simulink model "Dock_Charger"  (R2026b)
settings: Solver=VariableStepAuto
undefined symbols (not defined in the file or in its folder): P, Ts
libraries: nesl_utility x7, ee_lib x6, fl_lib x5, simulink x2, eeGeneralControl x1, batt_lib x1
settings Model: Creator=aomar  LastModifiedBy=aomar

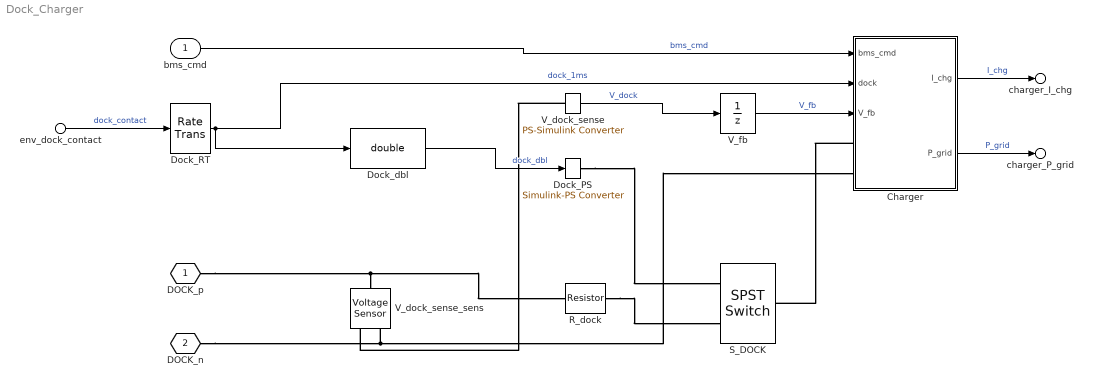
== system Dock_Charger ==
  bms_cmd : Inport  OutDataTypeStr=Bus: Bus_BMS_Cmd  SampleTime=Ts.bms_fast
  env_dock_contact : Inport  Port=2  PortName=env  Element=dock_contact
  Charger : Subsystem  Variant=on
  Dock_PS : nesl_utility/Simulink-PS Converter  PhysicalDomain=network_engine_domain  SubClassName=ps_input  LeftPortType=input  RightPortType=output  PseudoPeriodic=off  Frequencies=[]  NoiseDistribution=none  NoiseParameters=[]  Unit=V  AffineConversion=off  FilteringAndDerivatives=zero  SimscapeFilterOrder=1  InputFilterTimeConstant=0.001  UdotUserProvided=0
  Dock_RT : RateTransition  OutPortSampleTime=Ts.base
  Dock_dbl : DataTypeConversion  OutDataTypeStr=double  SaturateOnIntegerOverflow=off  RndMeth=Floor
  R_dock : ee_lib/Passive/Resistor  R=P.power.charger.R_dock Ohm  enable_R_tol=ee.enum.toleranceApplication.none  R_tol=5  tol_distribution=ee.enum.toleranceDistribution.uniform  nSigma=4  enable_operating_limits=ee.enum.enable.no  operating_limit_action=ee.enum.passive.reportOpLim.warn  power_rating=1 W  max_working_voltage=100 V  noise_mode=ee.enum.sources.noise.Disabled  Tdevice=25 degC  sample_time=1e-3 s  repeatability=ee.enum.ic.repeatability.notRepeatable  user_seed=0  auto_seed=1684602222  power_derating_T1=70 degC  power_derating_T2=155 degC  operating_temperature_range_vec=[-50, 150] degC  alpha=3.93e-3 1/K  Tmeas=25 degC  thermal_mass=100 J/K  temperature_specify=off  temperature_priority=High  temperature=298.15 K  temperature_nominal_specify=off  temperature_nominal_value=1  temperature_nominal_unit=K
  S_DOCK : ee_lib/Switches & Breakers/SPST Switch  R_closed=1e-6 Ohm  G_open=1e-8 S  Threshold=0.5 V  Width=0 V  model_dynamics=0  t_on=1e-3 s  t_off=1e-3 s  initial_vT=0 V
  V_dock_sense : nesl_utility/PS-Simulink Converter  PhysicalDomain=network_engine_domain  SubClassName=ps_output  LeftPortType=input  RightPortType=output  PseudoPeriodic=off  Frequencies=[]  VectorFormat=inherit  Unit=V  AffineConversion=off
  V_dock_sense_sens : fl_lib/Electrical/Electrical Sensors/Voltage Sensor
  V_fb : UnitDelay  SampleTime=Ts.base
  DOCK_p : PMIOPort  Side=Left  ConnectionType=Connection: foundation.electrical.electrical
  DOCK_n : PMIOPort  Port=2  Side=Left  ConnectionType=Connection: foundation.electrical.electrical
  charger_P_grid : Outport  PortName=charger  Element=P_grid
  charger_I_chg : Outport  PortName=charger  Element=I_chg
  wires:
  env_dock_contact/1 -> Dock_RT/1  "dock_contact"
  bms_cmd/1 -> Charger/1(bms_cmd)  "bms_cmd"
  Dock_RT/1 -> Charger/2(dock), Dock_dbl/1  "dock_1ms"
  Dock_dbl/1 -> Dock_PS/1  "dock_dbl"
  V_dock_sense/1 -> V_fb/1  "V_dock"
  V_fb/1 -> Charger/3(V_fb)  "V_fb"
  Charger/1(I_chg) -> charger_I_chg/1  "I_chg"
  Charger/2(P_grid) -> charger_P_grid/1  "P_grid"
  connections:
  Charger/LConn1 -- S_DOCK/RConn1
  V_dock_sense_sens/RConn2 -- DOCK_n/RConn1 -- Charger/LConn2
  V_dock_sense_sens/LConn1 -- DOCK_p/RConn1 -- R_dock/LConn1
  Dock_PS/RConn1 -- S_DOCK/LConn1
  R_dock/RConn1 -- S_DOCK/LConn2
  V_dock_sense/LConn1 -- V_dock_sense_sens/RConn1

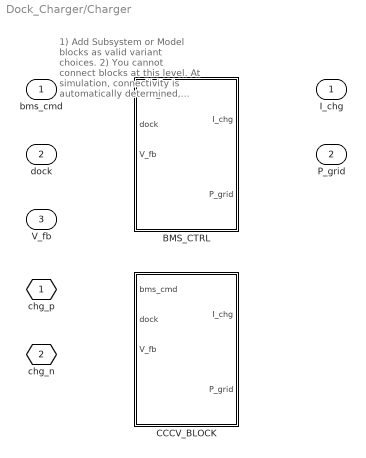
== system Dock_Charger/Charger ==
  note: 1) Add Subsystem or Model blocks as valid variant choices.
      | 2) You cannot connect blocks at this level. At simulation, connectivity is automatically
      | determined, based on the active variant and port name matching.
  bms_cmd : Inport
  dock : Inport  Port=2
  V_fb : Inport  Port=3
  BMS_CTRL : Subsystem  VariantControl=VC_CHG == 1
  CCCV_BLOCK : Subsystem  VariantControl=VC_CHG == 2
  chg_p : PMIOPort  Side=Left  ConnectionType=Connection: foundation.electrical.electrical
  chg_n : PMIOPort  Port=2  Side=Left  ConnectionType=Connection: foundation.electrical.electrical
  I_chg : Outport
  P_grid : Outport  Port=2

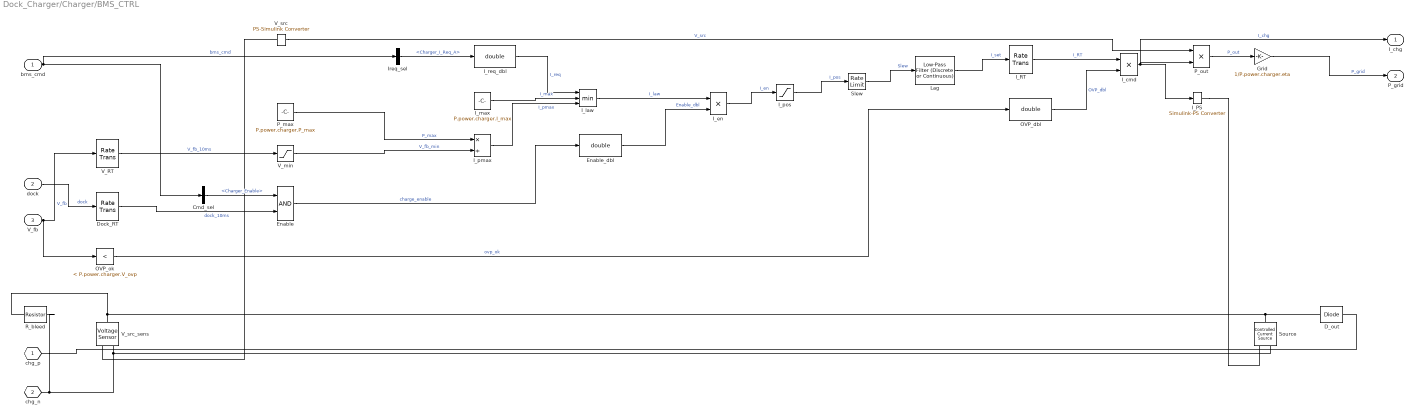
== system Dock_Charger/Charger/BMS_CTRL ==
  bms_cmd : Inport
  dock : Inport  Port=2
  V_fb : Inport  Port=3
  Cmd_sel : BusSelector  OutputSignals=Charger_Enable
  D_out : ee_lib/Semiconductors & Converters/Diode  Vf=P.power.charger.diode_Vf V  Ron=P.power.charger.diode_Ron Ohm  Goff=P.power.charger.diode_Goff S  N_series=1  N_parallel=1  ZenerEnable=false  BV=30 V  Rz=0.3 Ohm  enable_fault_composite=simscape.enum.onoff.off  i_specify=off  i_priority=None  i=0 A  i_nominal_specify=off  i_nominal_value=1  i_nominal_unit=A  v_specify=off  v_priority=None  v=0 V  v_nominal_specify=off  v_nominal_value=1  v_nominal_unit=V  ModelType=ee.enum.diode.idealModelType.pwl  TableType=ee.enum.diode.tableType.IfMat  IfMat=[.07, .12, .19, 1.75, 4.24, 7.32, 11.2; .16, .3, .72, 2.14, 5.02, 8.35, 13.12] A  VfMat=[.9, 1.15, 1.25, 1.5, 1.75, 2.17, 2.6, 2.85; .58, .68, .75, 1.1, 1.38, 1.77, 2.27, 2.7] V  TjVec=[25, 125] degC  VfVec=[.5, .7, .9, 1.3, 1.7, 2.1, 2.5] V  IfVec=[.1, .2, .5, 1, 2, 4, 7, 10] A  IrMat=[1e-06, 2e-06, 5e-06, 1e-05, 2.5e-05, 5e-05, .0001; 2e-06, 5e-06, 1e-05, 4e-05, 8e-05, .0002, .0005] A  VrMat=[10, 100, 200, 250, 300, 325, 350; 10, 70, 160, 220, 270, 300, 320] V  VrVec=[10, 20, 40, 50, 70, 80, 100] V  IrVec=[1e-06, 2e-06, 5e-06, 1e-05, 2e-05, 5e-05, .0001] A  rec_loss_model=ee.enum.diode.reverseRecoveryModelTabulateUpTo3D.fixed  ErecVal=0 J  scaleWithIandV=true  ErecMat=zeros(2, 3) J  ErecMat3D=zeros(2, 3, 2) J  TjrecVec=[25, 125] degC  IfrecVec=[.1, 1, 10] A  IrecVal=10 A  VrecVal=10 V  VrecVec=[0, 100] V  tFilter=1 / 1000 / 100 s  thermal_network_parameterization=ee.enum.thermalNetworkTopology.junctionCase  Rth=[0, 10] K/W  Rth_Cauer=[1, 3, 10] K/W  Rth_Foster=[.08, .14, .22, .16] K/W  thermal_mass_parameterization=ee.enum.thermalNetwork.timeconstant  thermal_mass=[0, 1] J/K  thermal_mass_Cauer=[.1, .3, 1] J/K  thermal_mass_Foster=[.001, .005, .05, .5] J/K  thermal_time_constant=[0, 10] s  thermal_time_constant_Cauer=[1, 3, 10] s  thermal_time_constant_Foster=[7e-05, .0007, .01, .08] s  thermal_mass_initial_temperatures=[25, 25] degC  thermal_mass_initial_temperatures_Cauer=[25, 25, 25] degC  thermal_mass_initial_temperatures_Foster=[25, 25, 25, 25] degC  junction_thermal_mass=0.01 J/K  junction_temperature_specify=off  junction_temperature_priority=None  junction_temperature=25 degC  junction_temperature_nominal_specify=off  junction_temperature_nominal_value=1  junction_temperature_nominal_unit=degC  ThermalPort=false  ModelTypePhysical=ee.enum.diode.physicalModelType.exponential  prmExp=ee.enum.diode.expParam.useTwo  I12=[.0137, .545] A  V12=[.6, .7] V  IS=1e-12 A  ec=1  I1=0.0137 A  V1=0.6 V  RS=0 Ohm  C_param=ee.enum.diode.capParam.fixed  CJ=0 pF  CJ0=5 pF  Vvec=[.1, 10, 100] V  Cvec=[3.5, 1, .4] pF  VJ=1 V  Mgrad=0.5  FC=0.5  Q_param=ee.enum.diode.recoveryParam.off  iRM=-7.15 A  iF=4 A  didt=-750 A/us  trr_factor=3  trr=115 ns  Qrr=150 nA*s  Vr=-600 V  Ls=150 nH  Erec=0.03 J  TT=50 ns  tau=100 ns  T_param=ee.enum.diode.temperatureParam.off  Tmeas=25 degC  I1_T2=0.245 A  V1_T2=0.5 V  IS_T2=1.25e-7 A  Tmeas2=125 degC  EG_param=ee.enum.diode.egapParam.material_si  EG=1.11 eV  XTI_param=ee.enum.diode.xtiParam.pn  XTI=3  dBVdT=0 V/K  Tdevice=25 degC  i_capacitor_specify=off  i_capacitor_priority=None  i_capacitor=0 A  i_capacitor_nominal_specify=off  i_capacitor_nominal_value=1  i_capacitor_nominal_unit=A  Qj_specify=off  Qj_priority=None  Qj=0 C  Qj_nominal_specify=off  Qj_nominal_value=1  Qj_nominal_unit=uC
  Dock_RT : RateTransition  OutPortSampleTime=Ts.bms_fast
  Enable : Logic  AllPortsSameDT=off  OutDataTypeStr=boolean
  Enable_dbl : DataTypeConversion  OutDataTypeStr=double  SaturateOnIntegerOverflow=off  RndMeth=Floor
  Grid : Gain  Gain=1/P.power.charger.eta
  I_PS : nesl_utility/Simulink-PS Converter  PhysicalDomain=network_engine_domain  SubClassName=ps_input  LeftPortType=input  RightPortType=output  PseudoPeriodic=off  Frequencies=[]  NoiseDistribution=none  NoiseParameters=[]  Unit=A  AffineConversion=off  FilteringAndDerivatives=zero  SimscapeFilterOrder=1  InputFilterTimeConstant=0.001  UdotUserProvided=0
  I_RT : RateTransition  OutPortSampleTime=Ts.base
  I_cmd : Product
  I_en : Product
  I_law : MinMax  Inputs=3
  I_max : Constant  Value=P.power.charger.I_max  SampleTime=Ts.bms_fast
  I_pmax : Product  Inputs=*/
  I_pos : Saturate  UpperLimit=inf  LowerLimit=0
  I_req_dbl : DataTypeConversion  OutDataTypeStr=double  SaturateOnIntegerOverflow=off  RndMeth=Floor
  Ireq_sel : BusSelector  OutputSignals=Charger_I_Req_A
  Lag : eeGeneralControl/Low-Pass Filter (Discrete or Continuous)  K=1  T=P.power.charger.tau  B=inf  A=-inf  init_option=Specify as parameter  x0=0  Ts=Ts.bms_fast
  OVP_dbl : DataTypeConversion  OutDataTypeStr=double  SaturateOnIntegerOverflow=off  RndMeth=Floor
  OVP_ok : simulink/Logic and Bit Operations/Compare To Constant  relop=<  const=P.power.charger.V_ovp  OutDataTypeStr=boolean
  P_max : Constant  Value=P.power.charger.P_max  SampleTime=Ts.bms_fast
  P_out : Product
  R_bleed : ee_lib/Passive/Resistor  R=P.power.charger.R_bleed Ohm  enable_R_tol=ee.enum.toleranceApplication.none  R_tol=5  tol_distribution=ee.enum.toleranceDistribution.uniform  nSigma=4  enable_operating_limits=ee.enum.enable.no  operating_limit_action=ee.enum.passive.reportOpLim.warn  power_rating=1 W  max_working_voltage=100 V  noise_mode=ee.enum.sources.noise.Disabled  Tdevice=25 degC  sample_time=1e-3 s  repeatability=ee.enum.ic.repeatability.notRepeatable  user_seed=0  auto_seed=2815256101  power_derating_T1=70 degC  power_derating_T2=155 degC  operating_temperature_range_vec=[-50, 150] degC  alpha=3.93e-3 1/K  Tmeas=25 degC  thermal_mass=100 J/K  temperature_specify=off  temperature_priority=High  temperature=298.15 K  temperature_nominal_specify=off  temperature_nominal_value=1  temperature_nominal_unit=K
  Slew : RateLimiter  RisingSlewLimit=P.power.charger.slew  FallingSlewLimit=-P.power.charger.slew  SampleTimeMode=inherited
  Source : fl_lib/Electrical/Electrical Sources/Controlled Current Source
  V_RT : RateTransition  OutPortSampleTime=Ts.bms_fast
  V_min : Saturate  UpperLimit=inf  LowerLimit=1
  V_src : nesl_utility/PS-Simulink Converter  PhysicalDomain=network_engine_domain  SubClassName=ps_output  LeftPortType=input  RightPortType=output  PseudoPeriodic=off  Frequencies=[]  VectorFormat=inherit  Unit=V  AffineConversion=off
  V_src_sens : fl_lib/Electrical/Electrical Sensors/Voltage Sensor
  chg_p : PMIOPort  Side=Left  ConnectionType=Connection: foundation.electrical.electrical
  chg_n : PMIOPort  Port=2  Side=Left  ConnectionType=Connection: foundation.electrical.electrical
  I_chg : Outport
  P_grid : Outport  Port=2
  wires:
  bms_cmd/1 -> Cmd_sel/1, Ireq_sel/1  "bms_cmd"
  dock/1 -> Dock_RT/1  "dock"
  V_fb/1 -> V_RT/1, OVP_ok/1  "V_fb"
  OVP_ok/1 -> OVP_dbl/1  "ovp_ok"
  V_RT/1 -> V_min/1  "V_fb_10ms"
  Dock_RT/1 -> Enable/2  "dock_10ms"
  Cmd_sel/1 -> Enable/1  "<Charger_Enable>"
  V_src/1 -> P_out/1  "V_src"
  P_max/1 -> I_pmax/1  "P_max"
  V_min/1 -> I_pmax/2  "V_fb_min"
  Enable/1 -> Enable_dbl/1  "charge_enable"
  Ireq_sel/1 -> I_req_dbl/1  "<Charger_I_Req_A>"
  I_max/1 -> I_law/2  "I_max"
  I_pmax/1 -> I_law/3  "I_pmax"
  I_req_dbl/1 -> I_law/1  "I_req"
  I_law/1 -> I_en/1  "I_law"
  Enable_dbl/1 -> I_en/2  "Enable_dbl"
  I_en/1 -> I_pos/1  "I_en"
  I_pos/1 -> Slew/1  "I_pos"
  Slew/1 -> Lag/1  "Slew"
  Lag/1 -> I_RT/1  "I_set"
  I_RT/1 -> I_cmd/1  "I_RT"
  OVP_dbl/1 -> I_cmd/2  "OVP_dbl"
  I_cmd/1 -> I_PS/1, I_chg/1, P_out/2  "I_chg"
  P_out/1 -> Grid/1  "P_out"
  Grid/1 -> P_grid/1  "P_grid"
  connections:
  V_src_sens/LConn1 -- R_bleed/LConn1 -- Source/LConn1 -- D_out/LConn1
  I_PS/RConn1 -- Source/RConn1
  V_src/LConn1 -- V_src_sens/RConn1
  chg_p/RConn1 -- D_out/RConn1
  chg_n/RConn1 -- R_bleed/RConn1 -- V_src_sens/RConn2 -- Source/RConn2

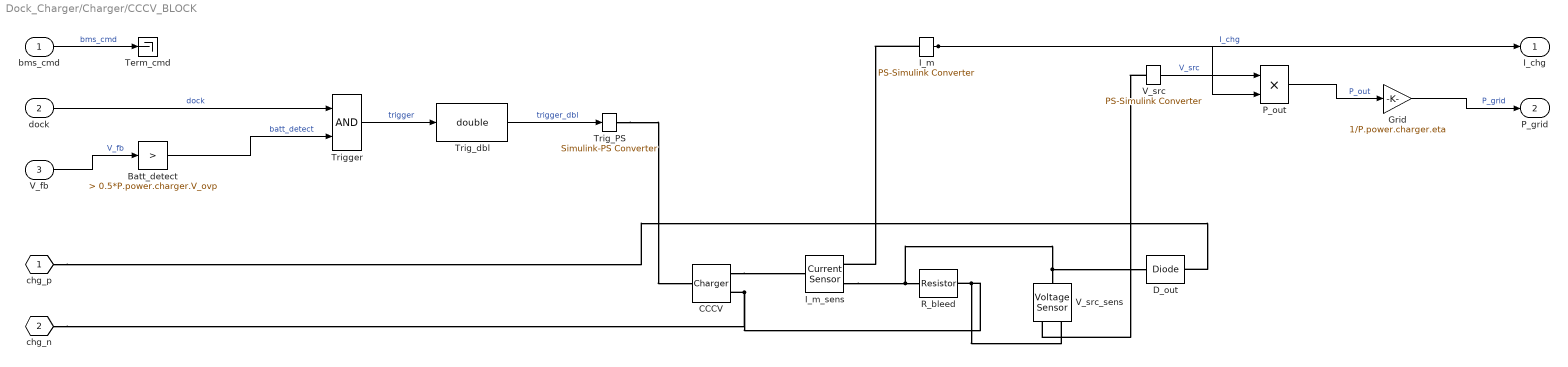
== system Dock_Charger/Charger/CCCV_BLOCK ==
  bms_cmd : Inport
  dock : Inport  Port=2
  V_fb : Inport  Port=3
  Batt_detect : simulink/Logic and Bit Operations/Compare To Constant  relop=>  const=0.5*P.power.charger.V_ovp  OutDataTypeStr=boolean
  CCCV : batt_lib/Cyclers/Charger  charging_current=P.power.charger.cccv_I A  voltage_threshold=P.power.charger.cccv_Vth V  charging_voltage=P.power.charger.cccv_V V  current_threshold=P.power.charger.cccv_Ith A
  D_out : ee_lib/Semiconductors & Converters/Diode  Vf=P.power.charger.diode_Vf V  Ron=P.power.charger.diode_Ron Ohm  Goff=P.power.charger.diode_Goff S  N_series=1  N_parallel=1  ZenerEnable=false  BV=30 V  Rz=0.3 Ohm  enable_fault_composite=simscape.enum.onoff.off  i_specify=off  i_priority=None  i=0 A  i_nominal_specify=off  i_nominal_value=1  i_nominal_unit=A  v_specify=off  v_priority=None  v=0 V  v_nominal_specify=off  v_nominal_value=1  v_nominal_unit=V  ModelType=ee.enum.diode.idealModelType.pwl  TableType=ee.enum.diode.tableType.IfMat  IfMat=[.07, .12, .19, 1.75, 4.24, 7.32, 11.2; .16, .3, .72, 2.14, 5.02, 8.35, 13.12] A  VfMat=[.9, 1.15, 1.25, 1.5, 1.75, 2.17, 2.6, 2.85; .58, .68, .75, 1.1, 1.38, 1.77, 2.27, 2.7] V  TjVec=[25, 125] degC  VfVec=[.5, .7, .9, 1.3, 1.7, 2.1, 2.5] V  IfVec=[.1, .2, .5, 1, 2, 4, 7, 10] A  IrMat=[1e-06, 2e-06, 5e-06, 1e-05, 2.5e-05, 5e-05, .0001; 2e-06, 5e-06, 1e-05, 4e-05, 8e-05, .0002, .0005] A  VrMat=[10, 100, 200, 250, 300, 325, 350; 10, 70, 160, 220, 270, 300, 320] V  VrVec=[10, 20, 40, 50, 70, 80, 100] V  IrVec=[1e-06, 2e-06, 5e-06, 1e-05, 2e-05, 5e-05, .0001] A  rec_loss_model=ee.enum.diode.reverseRecoveryModelTabulateUpTo3D.fixed  ErecVal=0 J  scaleWithIandV=true  ErecMat=zeros(2, 3) J  ErecMat3D=zeros(2, 3, 2) J  TjrecVec=[25, 125] degC  IfrecVec=[.1, 1, 10] A  IrecVal=10 A  VrecVal=10 V  VrecVec=[0, 100] V  tFilter=1 / 1000 / 100 s  thermal_network_parameterization=ee.enum.thermalNetworkTopology.junctionCase  Rth=[0, 10] K/W  Rth_Cauer=[1, 3, 10] K/W  Rth_Foster=[.08, .14, .22, .16] K/W  thermal_mass_parameterization=ee.enum.thermalNetwork.timeconstant  thermal_mass=[0, 1] J/K  thermal_mass_Cauer=[.1, .3, 1] J/K  thermal_mass_Foster=[.001, .005, .05, .5] J/K  thermal_time_constant=[0, 10] s  thermal_time_constant_Cauer=[1, 3, 10] s  thermal_time_constant_Foster=[7e-05, .0007, .01, .08] s  thermal_mass_initial_temperatures=[25, 25] degC  thermal_mass_initial_temperatures_Cauer=[25, 25, 25] degC  thermal_mass_initial_temperatures_Foster=[25, 25, 25, 25] degC  junction_thermal_mass=0.01 J/K  junction_temperature_specify=off  junction_temperature_priority=None  junction_temperature=25 degC  junction_temperature_nominal_specify=off  junction_temperature_nominal_value=1  junction_temperature_nominal_unit=degC  ThermalPort=false  ModelTypePhysical=ee.enum.diode.physicalModelType.exponential  prmExp=ee.enum.diode.expParam.useTwo  I12=[.0137, .545] A  V12=[.6, .7] V  IS=1e-12 A  ec=1  I1=0.0137 A  V1=0.6 V  RS=0 Ohm  C_param=ee.enum.diode.capParam.fixed  CJ=0 pF  CJ0=5 pF  Vvec=[.1, 10, 100] V  Cvec=[3.5, 1, .4] pF  VJ=1 V  Mgrad=0.5  FC=0.5  Q_param=ee.enum.diode.recoveryParam.off  iRM=-7.15 A  iF=4 A  didt=-750 A/us  trr_factor=3  trr=115 ns  Qrr=150 nA*s  Vr=-600 V  Ls=150 nH  Erec=0.03 J  TT=50 ns  tau=100 ns  T_param=ee.enum.diode.temperatureParam.off  Tmeas=25 degC  I1_T2=0.245 A  V1_T2=0.5 V  IS_T2=1.25e-7 A  Tmeas2=125 degC  EG_param=ee.enum.diode.egapParam.material_si  EG=1.11 eV  XTI_param=ee.enum.diode.xtiParam.pn  XTI=3  dBVdT=0 V/K  Tdevice=25 degC  i_capacitor_specify=off  i_capacitor_priority=None  i_capacitor=0 A  i_capacitor_nominal_specify=off  i_capacitor_nominal_value=1  i_capacitor_nominal_unit=A  Qj_specify=off  Qj_priority=None  Qj=0 C  Qj_nominal_specify=off  Qj_nominal_value=1  Qj_nominal_unit=uC
  Grid : Gain  Gain=1/P.power.charger.eta
  I_m : nesl_utility/PS-Simulink Converter  PhysicalDomain=network_engine_domain  SubClassName=ps_output  LeftPortType=input  RightPortType=output  PseudoPeriodic=off  Frequencies=[]  VectorFormat=inherit  Unit=A  AffineConversion=off
  I_m_sens : fl_lib/Electrical/Electrical Sensors/Current Sensor
  P_out : Product
  R_bleed : ee_lib/Passive/Resistor  R=P.power.charger.R_bleed Ohm  enable_R_tol=ee.enum.toleranceApplication.none  R_tol=5  tol_distribution=ee.enum.toleranceDistribution.uniform  nSigma=4  enable_operating_limits=ee.enum.enable.no  operating_limit_action=ee.enum.passive.reportOpLim.warn  power_rating=1 W  max_working_voltage=100 V  noise_mode=ee.enum.sources.noise.Disabled  Tdevice=25 degC  sample_time=1e-3 s  repeatability=ee.enum.ic.repeatability.notRepeatable  user_seed=0  auto_seed=735241226  power_derating_T1=70 degC  power_derating_T2=155 degC  operating_temperature_range_vec=[-50, 150] degC  alpha=3.93e-3 1/K  Tmeas=25 degC  thermal_mass=100 J/K  temperature_specify=off  temperature_priority=High  temperature=298.15 K  temperature_nominal_specify=off  temperature_nominal_value=1  temperature_nominal_unit=K
  Term_cmd : Terminator
  Trig_PS : nesl_utility/Simulink-PS Converter  PhysicalDomain=network_engine_domain  SubClassName=ps_input  LeftPortType=input  RightPortType=output  PseudoPeriodic=off  Frequencies=[]  NoiseDistribution=none  NoiseParameters=[]  Unit=1  AffineConversion=off  FilteringAndDerivatives=zero  SimscapeFilterOrder=1  InputFilterTimeConstant=0.001  UdotUserProvided=0
  Trig_dbl : DataTypeConversion  OutDataTypeStr=double  SaturateOnIntegerOverflow=off  RndMeth=Floor
  Trigger : Logic  AllPortsSameDT=off  OutDataTypeStr=boolean
  V_src : nesl_utility/PS-Simulink Converter  PhysicalDomain=network_engine_domain  SubClassName=ps_output  LeftPortType=input  RightPortType=output  PseudoPeriodic=off  Frequencies=[]  VectorFormat=inherit  Unit=V  AffineConversion=off
  V_src_sens : fl_lib/Electrical/Electrical Sensors/Voltage Sensor
  chg_p : PMIOPort  Side=Left  ConnectionType=Connection: foundation.electrical.electrical
  chg_n : PMIOPort  Port=2  Side=Left  ConnectionType=Connection: foundation.electrical.electrical
  I_chg : Outport
  P_grid : Outport  Port=2
  wires:
  bms_cmd/1 -> Term_cmd/1  "bms_cmd"
  dock/1 -> Trigger/1  "dock"
  V_fb/1 -> Batt_detect/1  "V_fb"
  Batt_detect/1 -> Trigger/2  "batt_detect"
  Trigger/1 -> Trig_dbl/1  "trigger"
  Trig_dbl/1 -> Trig_PS/1  "trigger_dbl"
  I_m/1 -> P_out/2, I_chg/1  "I_chg"
  V_src/1 -> P_out/1  "V_src"
  P_out/1 -> Grid/1  "P_out"
  Grid/1 -> P_grid/1  "P_grid"
  connections:
  Trig_PS/RConn1 -- CCCV/LConn1
  CCCV/RConn1 -- I_m_sens/LConn1
  CCCV/RConn2 -- chg_n/RConn1 -- R_bleed/RConn1 -- V_src_sens/RConn2
  R_bleed/LConn1 -- I_m_sens/RConn2 -- V_src_sens/LConn1 -- D_out/LConn1
  chg_p/RConn1 -- D_out/RConn1
  I_m/LConn1 -- I_m_sens/RConn1
  V_src/LConn1 -- V_src_sens/RConn1
